simulink model "BoostPFCConverter"  (R2026a)
settings: Solver=ode23t  StopTime=0.05  MaxStep=1e-5  AbsTol=1e-3
PreLoadFcn:
  | BoostPFCDefaultInputParameters;
model workspace (MAT data in the model file):
  ConverterKey : string (value not decoded)
undefined symbols (not defined in the file): boostPFCController, boostPFCDesign, Rload_R, Vref
libraries: fl_lib x27, ee_lib x14, nesl_utility x14, ConverterLibrary x1
(part 2 of 2)

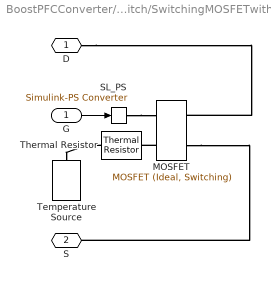
== system BoostPFCConverter/Boost PFC/BoostPFCVariant/DetailedModel/BoostSwitch/SwitchingMOSFETwithThermal ==
  G : Inport
  MOSFET : ee_lib/Semiconductors & Converters/MOSFET (Ideal, Switching)  PartSpecification="{\"CollectionId\":\"MW.SimscapeElectrical\",\"CollectionVersion\":\"1.0.0\",\"DatasetId\":\"Wolfspeed|C3M0015065K|\",\"DisplayName\":\"Wolfspeed:C3M0015065K\"}"  port_option=ee.enum.controlport.ps  Rds=0.015 % Datasheet derived Ohm  Goff=1.53846153846154e-09 % Datasheet derived S  Vth=2.3 % Wolfspeed XML derived V  diode_param=ee.enum.semiconductors.protectionDiode.external  diode_Vf=1.96 % Datasheet derived V  diode_Ron=0.007 % Wolfspeed XML derived Ohm  diode_Goff=1e-05 % Library default S  diode_C=50e-9 % Parameter not set F  diode_iRM=-235 % Parameter not set A  diode_iF=300 % Parameter not set A  diode_idot=-50 % Parameter not set A/us  diode_trr_param=ee.enum.converters.diodeReverseParam.trr_factor  diode_trr_factor=3 % Parameter not set  diode_trr=15 % Parameter not set us  diode_Qrr=1500 % Parameter not set s*uA  ids_specify=off  ids_priority=None  ids=0 A  ids_nominal_specify=off  ids_nominal_value=1  ids_nominal_unit=A  vds_specify=off  vds_priority=None  vds=0 V  vds_nominal_specify=off  vds_nominal_value=1  vds_nominal_unit=V  vgs_specify=off  vgs_priority=None  vgs=0 V  vgs_nominal_specify=off  vgs_nominal_value=1  vgs_nominal_unit=V  thermal_loss_option=ee.enum.converters.thermalLossOption.tabulated2d  Von_data=[-2.66 -2.44 -1.95 -1.414 -0.78 -0.41 -0.165 -0.082 -0.0343 0 0.037 0.078 0.179 0.43 0.83 1.68 2.597 3.5358 4.01;-2.83 -2.54 -1.975 -1.397 -0.75 -0.38 -0.155 -0.08 -0.03 0 0.034 0.067 0.16 0.39 0.76 1.549 2.4 3.26 3.72;-4.517 -4 -2.934 -1.965 -1 -0.51 -0.2048 -0.1018 -0.041 0 0.042 0.085 0.2 0.496 0.997 2.035 3.12 4.4 5.045;-5 -4.4 -3.2274 -2.1615 -1.1 -0.561 -0.22528 -0.11198 -0.0451 0 0.0462 0.0935 0.22 0.5456 1.0967 2.2385 3.432 4.84 5.5495] % Wolfspeed XML derived V  Tj=[-40 25 175 900] % Wolfspeed XML derived degC  Iout_data=[-225 -200 -150 -100 -50 -25 -10 -5 -2 0 2 5 10 25 50 100 150 200 225] % Wolfspeed XML derived A  tabulateWithVds=true  Eon_data=[0 9.96967576216216e-05 0.000145936917654886 0.000196497951068607 0.00019967532764657 0.000247335976316008 0.000304217502237006 0.000365133507991684;0 9.59855482079002e-05 0.000143792560765073 0.000194828655567568 0.000198273960318087 0.000249953531575884 0.000309139293804574 0.000373083909954262;0 9.79543049313929e-05 0.00014827399604158 0.000204722913230769 0.000208316887241164 0.000262226497397089 0.000326590011941788 0.000392096453887734;0 9.94356283409563e-05 0.000153658587442827 0.000209975271517672 0.000213824500004158 0.000271562927301455 0.000335992545829522 0.000402717496316008;0 0.000104407409862786 0.000161341516640333 0.000220474035093555 0.000224515725 0.000285141073596674 0.000352792173505198 0.000422853371376299] % Wolfspeed XML derived J  Eoff_data=[0 1.84408651719851e-05 4.70462491740572e-05 8.90430247881139e-05 9.1842809829051e-05 0.000147567719056776 0.000209864407870079 0.000278943613503315;0 2.00265752898881e-05 4.98845677374637e-05 9.33904774060557e-05 9.62908713839619e-05 0.000152525717421674 0.000215755778797141 0.000286903323875052;0 1.96758643514298e-05 5.11710664647741e-05 9.55627110851896e-05 9.8522154059884e-05 0.000155956102939287 0.000220242998240779 0.000292319989582884;0 1.96080415026937e-05 5.1490482059884e-05 9.66068334349875e-05 9.96145901933278e-05 0.000157442558060298 0.000223828680222752 0.000296440030520307;0 2.05884438265644e-05 5.40650061317862e-05 0.000101437175308835 0.000104595319920638 0.000165314685994405 0.000235020113767509 0.00031126203170431] % Wolfspeed XML derived J  Eon_data_3D=reshape([0;0;0;0;0;0;0;0;0;0;0;0;0;0;0;0;0;0;0;0;0;0;0;0;0;0;0;0;0;0;0;0;0;0;0;0;0;0;0;0;0;0;0;0;0;0;0;0;0;0;0;0;0;0;0;0;0;0;0;0;0;0;0;0;0;0;0;0;0;0;0;0;0;0;0;0;0;0;0;0;0;0;0;0;0;9.96967576216216e-05;9.59855482079002e-05;9.79543049313929e-05;9.94356283409563e-05;0.000104407409862786;0.000145936917654886;0.000143792560765073;0.00014827399604158;0.000153658587442827;0.000161341516640333;0.000196497951068607;0.000194828655567568;0.000204722913230769;0.000209975271517672;0.000220474035093555;0.00019967532764657;0.000198273960318087;0.000208316887241164;0.000213824500004158;0.000224515725;0.000247335976316008;0.000249953531575884;0.000262226497397089;0.000271562927301455;0.000285141073596674;0.000304217502237006;0.000309139293804574;0.000326590011941788;0.000335992545829522;0.000352792173505198;0.000365133507991684;0.000373083909954262;0.000392096453887734;0.000402717496316008;0.000422853371376299],[5 8 3]) % Wolfspeed XML derived J  Eoff_data_3D=reshape([0;0;0;0;0;0;0;0;0;0;0;0;0;0;0;0;0;0;0;0;0;0;0;0;0;0;0;0;0;0;0;0;0;0;0;0;0;0;0;0;0;0;0;0;0;0;0;0;0;0;0;0;0;0;0;0;0;0;0;0;0;0;0;0;0;0;0;0;0;0;0;0;0;0;0;0;0;0;0;0;0;0;0;0;0;1.84408651719851e-05;2.00265752898881e-05;1.96758643514298e-05;1.96080415026937e-05;2.05884438265644e-05;4.70462491740572e-05;4.98845677374637e-05;5.11710664647741e-05;5.1490482059884e-05;5.40650061317862e-05;8.90430247881139e-05;9.33904774060557e-05;9.55627110851896e-05;9.66068334349875e-05;0.000101437175308835;9.1842809829051e-05;9.62908713839619e-05;9.8522154059884e-05;9.96145901933278e-05;0.000104595319920638;0.000147567719056776;0.000152525717421674;0.000155956102939287;0.000157442558060298;0.000165314685994405;0.000209864407870079;0.000215755778797141;0.000220242998240779;0.000223828680222752;0.000235020113767509;0.000278943613503315;0.000286903323875052;0.000292319989582884;0.000296440030520307;0.00031126203170431],[5 8 3]) % Wolfspeed XML derived J  Tj_loss=[25 75 125 150 900] % Wolfspeed XML derived degC  Iout_data_loss=[0 12.8 26.4 38.4 39.2 51.2 62.4 74.4] % Wolfspeed XML derived A  Vds_loss=[-10 0 400] % Wolfspeed XML derived V  Eon_scalar=22.86e-3 % Parameter not set J  Eoff_scalar=17.14e-3 % Parameter not set J  Voff=300 % Parameter not set V  Iout_scalar=600 % Parameter not set A  useCurrentFromPreviousCycle=false % Parameter not set  useVoltageFromPreviousCycle=false % Parameter not set  diodeModelType=ee.enum.converters.diodeModelType.tabulated  diodeTableType=ee.enum.diode.tableType.VfMat  diode_ReverseIVType=ee.enum.diode.diodeReverseIV.constant  diode_IfMat=[.07, .12, .19, 1.75, 4.24, 7.32, 11.2; .16, .3, .72, 2.14, 4.02, 6.35, 9.12] % Parameter not set A  diode_VfMat=[0 2.87 3.94 4.34 5.07 5.76 6.58 7.12 7.53 7.697;0 2.68 3.54 3.9 4.55 5.26 6.12 6.72 7.18 7.38;0 2.31 3.11 3.45 4.06 4.72 5.61 6.24 6.76 6.987;0 2.079 2.799 3.105 3.654 4.248 5.049 5.616 6.084 6.3] % Wolfspeed XML derived V  diode_TjVec=[-40 25 175 900] % Wolfspeed XML derived degC  diode_VfVec=[.5, .7, .9, 1.3, 1.7, 2.1, 2.5] % Parameter not set V  diode_IfVec=[0 0.13 5 10 25 50 100 150 200 225] % Wolfspeed XML derived A  diode_IrMat=[1e-06, 2e-06, 5e-06, 1e-05, 2.5e-05, 5e-05, .0001; 2e-06, 5e-06, 1e-05, 4e-05, 8e-05, .0002, .0005] % Parameter not set A  diode_VrMat=[10, 100, 200, 250, 300, 325, 350; 10, 70, 160, 220, 270, 300, 320] % Parameter not set V  diode_VrVec=[10, 20, 40, 50, 70, 80, 100] % Parameter not set V  diode_IrVec=[1e-06, 2e-06, 5e-06, 1e-05, 2e-05, 5e-05, .0001] % Parameter not set A  diode_Vr=-600 % Parameter not set V  diode_Ls=150 % Parameter not set nH  diode_Erec=0.03 % Parameter not set J  diode_rec_loss_model=ee.enum.diode.reverseRecoveryModel.tabulated2d  diode_ErecVal=0 % Parameter not set J  diode_scaleWithIandV=true % Parameter not set  diode_ErecMat=[0 0;0 0] % Wolfspeed XML derived J  diodeErecMat3D=zeros(2, 3, 2) J  diode_TjrecVec=[25 35] % Wolfspeed XML derived degC  diode_IfrecVec=[0 10] % Wolfspeed XML derived A  diodeVrecVec=[0, 100] V  diode_IrecVal=10 % Parameter not set A  diode_VrecVal=10 % Wolfspeed XML derived V  diode_tFilter=1 / 1000 / 100 % Parameter not set s  separateThermalPortForDiode=false  thermal_network_parameterization=ee.enum.thermalNetworkTopology.external  Rth=[.03, .2] % Parameter not set K/W  Rth_Cauer=[0.040544078 0.111521813 0.073003418 0.124838849] % Wolfspeed XML derived K/W  Rth_Foster=[.08, .14, .22, .16] % Parameter not set K/W  thermal_mass_parameterization=ee.enum.thermalNetwork.thermalmass  thermal_mass=[3, 25] % Parameter not set J/K  thermal_mass_Cauer=[0.002121535 0.01054405 0.031037314 0.127325435] % Wolfspeed XML derived J/K  thermal_mass_Foster=[.001, .005, .05, .5] % Parameter not set J/K  thermal_time_constant=[.1, 5] % Parameter not set s  thermal_time_constant_Cauer=[.1, 1, 5] % Parameter not set s  thermal_time_constant_Foster=[7e-05, .0007, .01, .08] % Parameter not set s  thermal_mass_initial_temperatures=[25, 25] % Parameter not set degC  thermal_mass_initial_temperatures_Cauer=[25 25 25 25] % Wolfspeed XML derived degC  junction_thermal_mass=0.01 % Parameter not set J/K  Tvec_initial_Foster=[25, 25, 25, 25] % Parameter not set degC  RthDiode=[.03, .2] % Parameter not set K/W  RthCauerDiode=[0.04054 0.1115 0.073 0.1248] % Wolfspeed XML derived K/W  RthFosterDiode=[.03, .2] % Parameter not set K/W  thermalMassDiode=[3, 25] % Parameter not set J/K  thermalMassCauerDiode=[0.002122 0.01054 0.03104 0.1273] % Wolfspeed XML derived J/K  thermalMassFosterDiode=[33, 50] % Parameter not set J/K  thermalTauDiode=[.1, 5] % Parameter not set s  thermalTauCauerDiode=[.1, 1, 5] % Parameter not set s  thermalTauFosterDiode=[1, 10] % Parameter not set s  thermalMassInitTempDiode=[25, 25] % Parameter not set degC  thermalMassInitTempCauerDiode=[25 25 25 25] % Wolfspeed XML derived degC  junctionthermalMassDiode=0.1 % Parameter not set J/K  TVecInitialFosterDiode=[25, 25, 25, 25] % Parameter not set degC  no_thermal_network=0 % Parameter not set  mosfet_junction_temperature_specify=off  mosfet_junction_temperature_priority=None  mosfet_junction_temperature=simTemp_K K  mosfet_junction_temperature_nominal_specify=off  mosfet_junction_temperature_nominal_value=1  mosfet_junction_temperature_nominal_unit=degC  diode_junction_temperature_specify=off  diode_junction_temperature_priority=None  diode_junction_temperature=simTemp_K K  diode_junction_temperature_nominal_specify=off  diode_junction_temperature_nominal_value=1  diode_junction_temperature_nominal_unit=degC  Qj_specify=off  Qj_priority=None  Qj=0 W  Qj_nominal_specify=off  Qj_nominal_value=1  Qj_nominal_unit=W  accumulatedSwitchingLosses_specify=off  accumulatedSwitchingLosses_priority=None  accumulatedSwitchingLosses=0 J
      settings: AttributesFormatString=Wolfspeed:C3M0015065K
  SL_PS : nesl_utility/Simulink-PS Converter  PhysicalDomain=network_engine_domain  SubClassName=ps_input  LeftPortType=input  RightPortType=output  PseudoPeriodic=off  Frequencies=[]  NoiseDistribution=none  NoiseParameters=[]  Unit=1  AffineConversion=off  FilteringAndDerivatives=provide  SimscapeFilterOrder=1  InputFilterTimeConstant=0.001  UdotUserProvided=0
  Temperature Source : fl_lib/Thermal/Thermal Sources/Temperature Source  temperature=simTemp_K K
  Thermal Resistor : ee_lib/Passive/Thermal/Thermal Resistor  R=1e-3 K/W  T_specify=off  T_priority=None  T=0 K  T_nominal_specify=off  T_nominal_value=1  T_nominal_unit=K  Q_specify=off  Q_priority=None  Q=0 W  Q_nominal_specify=off  Q_nominal_value=1  Q_nominal_unit=W
  D : PMIOPort  Side=Left
  S : PMIOPort  Port=2  Side=Right
  wires:
  G/1 -> SL_PS/1
  connections:
  Thermal Resistor/LConn1 -- Temperature Source/LConn1
  MOSFET/LConn2 -- Thermal Resistor/RConn1
  MOSFET/RConn2 -- S/RConn1
  D/RConn1 -- MOSFET/RConn1
  SL_PS/RConn1 -- MOSFET/LConn1

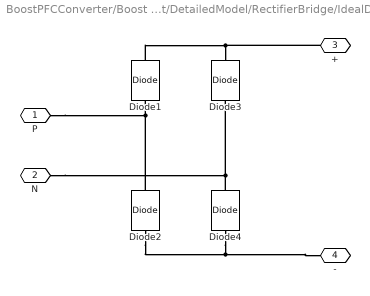
== system BoostPFCConverter/Boost PFC/BoostPFCVariant/DetailedModel/RectifierBridge/IdealDiode ==
  Diode{1..4} (4 alike) : fl_lib/Electrical/Electrical Elements/Diode  Vf=VfRect_SI V  Ron=RdRect_SI Ohm  Goff=GdRect_SI 1/Ohm  i_specify=off  i_priority=None  i=0 A  i_nominal_specify=off  i_nominal_value=1  i_nominal_unit=A  v_specify=off  v_priority=None  v=0 V  v_nominal_specify=off  v_nominal_value=1  v_nominal_unit=V
  P : PMIOPort  Side=Left
  N : PMIOPort  Port=2  Side=Left
  + : PMIOPort  Port=3  Side=Right
  - : PMIOPort  Port=4  Side=Right
  connections:
  Diode2/LConn1 -- -/RConn1 -- Diode4/LConn1
  Diode4/RConn1 -- N/RConn1 -- Diode3/LConn1
  Diode2/RConn1 -- P/RConn1 -- Diode1/LConn1
  Diode1/RConn1 -- +/RConn1 -- Diode3/RConn1

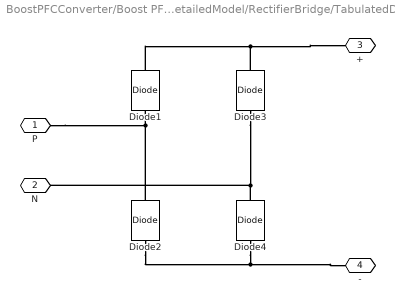
== system BoostPFCConverter/Boost PFC/BoostPFCVariant/DetailedModel/RectifierBridge/TabulatedDiode ==
  Diode1 : ee_lib/Semiconductors & Converters/Diode  PartSpecification="{\"CollectionId\":\"MW.SimscapeElectrical\",\"CollectionVersion\":\"1.0.0\",\"DatasetId\":\"Infineon|IDW80C65D1|simscape.electrical.diode\",\"DisplayName\":\"Infineon:IDW80C65D1\"}"  ModelType=ee.enum.diode.modelType.tabulated  TableType=ee.enum.diode.tableType.IfMat  IfMat=[0.0001 0.0001 0.1601 0.6065 1.9426 5.4603 12.2546 21.9425 34.4556 49.1982 64.7538 83.3404;0.3114 0.8503 2.3479 5.2232 9.8335 15.9488 23.5801 32.5233 43.1998 54.3228 66.653 79.8979] % Datasheet derived A  VfMat=[.9, 1.15, 1.25, 1.5, 1.75, 2.17, 2.6, 2.85; .58, .68, .75, 1.1, 1.38, 1.77, 2.27, 2.7] % Parameter not set V  TjVec=[25 175] % Datasheet derived degC  VfVec=[0.3258 0.4465 0.5672 0.6878 0.8085 0.9292 1.0498 1.1705 1.2912 1.4118 1.5325 1.6532] % Datasheet derived V  IfVec=[.1, .2, .5, 1, 2, 4, 7, 10] % Parameter not set A  IrMat=[1e-06, 2e-06, 5e-06, 1e-05, 2.5e-05, 5e-05, .0001; 2e-06, 5e-06, 1e-05, 4e-05, 8e-05, .0002, .0005] % Parameter not set A  VrMat=[10, 100, 200, 250, 300, 325, 350; 10, 70, 160, 220, 270, 300, 320] % Parameter not set V  VrVec=[10, 20, 40, 50, 70, 80, 100] % Parameter not set V  IrVec=[1e-06, 2e-06, 5e-06, 1e-05, 2e-05, 5e-05, .0001] % Parameter not set A  Vf=0.6 % Parameter not set V  Ron=0.3 % Parameter not set Ohm  Goff=1e-08 % Parameter not set S  prmExp=ee.enum.diode.expParam.useTwo  I12=[.0137, .545] % Parameter not set A  V12=[.6, .7] % Parameter not set V  RS=0 % Parameter not set Ohm  Tmeas=298.15 % Parameter not set K  IS=1e-12 % Parameter not set A  ec=1 % Parameter not set  I1=0.0137 % Parameter not set A  V1=0.6 % Parameter not set V  N_series=1 % Parameter not set  N_parallel=1 % Parameter not set  ZenerEnable=false % Parameter not set  Rz=0.3 % Parameter not set Ohm  BV=inf % Parameter not set V  C_param=ee.enum.diode.capParam.fixed  CJ=0 % Parameter not set pF  CJ0=5 % Parameter not set pF  Vvec=[.1, 10, 100] % Parameter not set V  Cvec=[3.5, 1, .4] % Parameter not set pF  VJ=1 % Parameter not set V  Mgrad=0.5 % Parameter not set  FC=0.5 % Parameter not set  Q_param=ee.enum.diode.recoveryParam.off  iRM=-7.15 % Parameter not set A  iF=4 % Parameter not set A  didt=-750 % Parameter not set A/us  trr_factor=3 % Parameter not set  trr=115 % Parameter not set ns  Qrr=150 % Parameter not set nA*s  Vr=-600 % Parameter not set V  Ls=150 % Parameter not set nH  Erec=0.03 % Parameter not set J  TT=50 % Parameter not set ns  tau=100 % Parameter not set ns  T_param=ee.enum.diode.temperatureParam.off  Tdevice=simTemp_K K  I1_T2=0.245 % Parameter not set A  V1_T2=0.5 % Parameter not set V  IS_T2=1.25e-7 % Parameter not set A  Tmeas2=125 % Parameter not set degC  XTI_param=ee.enum.diode.xtiParam.pn  XTI=3 % Parameter not set  EG_param=ee.enum.diode.egapParam.material_si  EG=1.11 % Parameter not set eV  dBVdT=0 % Parameter not set V/K  enable_fault_input=simscape.enum.onoff.off  i_specify=off  i_priority=None  i=0 A  i_nominal_specify=off  i_nominal_value=1  i_nominal_unit=A  v_specify=off  v_priority=None  v=0 V  v_nominal_specify=off  v_nominal_value=1  v_nominal_unit=V  v_capacitor_specify=off  v_capacitor_priority=None  v_capacitor=0 V  v_capacitor_nominal_specify=off  v_capacitor_nominal_value=1  v_capacitor_nominal_unit=V  Qj_specify=off  Qj_priority=High  Qj=0 C  Qj_nominal_specify=off  Qj_nominal_value=1  Qj_nominal_unit=C  i_diode_specify=off  i_diode_priority=None  i_diode=0 A  i_diode_nominal_specify=off  i_diode_nominal_value=1  i_diode_nominal_unit=A  v_diode_specify=off  v_diode_priority=None  v_diode=0 V  v_diode_nominal_specify=off  v_diode_nominal_value=1  v_diode_nominal_unit=V  i_capacitor_specify=off  i_capacitor_priority=None  i_capacitor=0 A  i_capacitor_nominal_specify=off  i_capacitor_nominal_value=1  i_capacitor_nominal_unit=A  fidelity_level=ee.enum.diode.fidelity.includeChargeDyn  rec_loss_model=ee.enum.diode.reverseRecoveryModel.fixed  ErecVal=0 % Parameter not set J  scaleWithIandV=true % Parameter not set  ErecMat=zeros(2, 3) % Parameter not set J  ErecMat3D=zeros(2, 3, 2) J  TjrecVec=[298.15, 398.15] % Parameter not set K  IfrecVec=[.1, 1, 10] % Parameter not set A  IrecVal=10 % Parameter not set A  VrecVal=10 % Parameter not set V  VrecVec=[0, 100] V  tFilter=1 / 1000 / 100 % Parameter not set s  thermal_network_parameterization=ee.enum.thermalNetworkTopology.junctionCase  Rth=[0, 10] % Parameter not set K/W  Rth_Cauer=[1, 3, 10] % Parameter not set K/W  Rth_Foster=[.08, .14, .22, .16] % Parameter not set K/W  thermal_mass_parameterization=ee.enum.thermalNetwork.timeconstant  thermal_mass=[0, 1] % Parameter not set J/K  thermal_mass_Cauer=[.1, .3, 1] % Parameter not set J/K  thermal_mass_Foster=[.001, .005, .05, .5] % Parameter not set J/K  thermal_time_constant=[0, 10] % Parameter not set s  thermal_time_constant_Cauer=[1, 3, 10] % Parameter not set s  thermal_time_constant_Foster=[7e-05, .0007, .01, .08] % Parameter not set s  thermal_mass_initial_temperatures=[25, 25] % Parameter not set degC  thermal_mass_initial_temperatures_Cauer=[25, 25, 25] % Parameter not set degC  junction_thermal_mass=0.01 % Parameter not set J/K  Tvec_initial_Foster=[25, 25, 25, 25] % Parameter not set degC  no_thermal_network=0 % Parameter not set  junction_temperature_specify=off  junction_temperature_priority=None  junction_temperature=25 degC  junction_temperature_nominal_specify=off  junction_temperature_nominal_value=1  junction_temperature_nominal_unit=degC
      settings: AttributesFormatString=Infineon:IDW80C65D1
  Diode2 : ee_lib/Semiconductors & Converters/Diode  ModelType=ee.enum.diode.modelType.tabulated  TableType=ee.enum.diode.tableType.IfMat  IfMat=[0.0001 0.0001 0.1601 0.6065 1.9426 5.4603 12.2546 21.9425 34.4556 49.1982 64.7538 83.3404;0.3114 0.8503 2.3479 5.2232 9.8335 15.9488 23.5801 32.5233 43.1998 54.3228 66.653 79.8979] % Datasheet derived A  VfMat=[.9, 1.15, 1.25, 1.5, 1.75, 2.17, 2.6, 2.85; .58, .68, .75, 1.1, 1.38, 1.77, 2.27, 2.7] % Parameter not set V  TjVec=[25 175] % Datasheet derived degC  VfVec=[0.3258 0.4465 0.5672 0.6878 0.8085 0.9292 1.0498 1.1705 1.2912 1.4118 1.5325 1.6532] % Datasheet derived V  IfVec=[.1, .2, .5, 1, 2, 4, 7, 10] % Parameter not set A  IrMat=[1e-06, 2e-06, 5e-06, 1e-05, 2.5e-05, 5e-05, .0001; 2e-06, 5e-06, 1e-05, 4e-05, 8e-05, .0002, .0005] % Parameter not set A  VrMat=[10, 100, 200, 250, 300, 325, 350; 10, 70, 160, 220, 270, 300, 320] % Parameter not set V  VrVec=[10, 20, 40, 50, 70, 80, 100] % Parameter not set V  IrVec=[1e-06, 2e-06, 5e-06, 1e-05, 2e-05, 5e-05, .0001] % Parameter not set A  Vf=0.6 % Parameter not set V  Ron=0.3 % Parameter not set Ohm  Goff=1e-08 % Parameter not set S  prmExp=ee.enum.diode.expParam.useTwo  I12=[.0137, .545] % Parameter not set A  V12=[.6, .7] % Parameter not set V  RS=0 % Parameter not set Ohm  Tmeas=298.15 % Parameter not set K  IS=1e-12 % Parameter not set A  ec=1 % Parameter not set  I1=0.0137 % Parameter not set A  V1=0.6 % Parameter not set V  N_series=1 % Parameter not set  N_parallel=1 % Parameter not set  ZenerEnable=false % Parameter not set  Rz=0.3 % Parameter not set Ohm  BV=inf % Parameter not set V  C_param=ee.enum.diode.capParam.fixed  CJ=0 % Parameter not set pF  CJ0=5 % Parameter not set pF  Vvec=[.1, 10, 100] % Parameter not set V  Cvec=[3.5, 1, .4] % Parameter not set pF  VJ=1 % Parameter not set V  Mgrad=0.5 % Parameter not set  FC=0.5 % Parameter not set  Q_param=ee.enum.diode.recoveryParam.off  iRM=-7.15 % Parameter not set A  iF=4 % Parameter not set A  didt=-750 % Parameter not set A/us  trr_factor=3 % Parameter not set  trr=115 % Parameter not set ns  Qrr=150 % Parameter not set nA*s  Vr=-600 % Parameter not set V  Ls=150 % Parameter not set nH  Erec=0.03 % Parameter not set J  TT=50 % Parameter not set ns  tau=100 % Parameter not set ns  T_param=ee.enum.diode.temperatureParam.off  Tdevice=simTemp_K K  I1_T2=0.245 % Parameter not set A  V1_T2=0.5 % Parameter not set V  IS_T2=1.25e-7 % Parameter not set A  Tmeas2=125 % Parameter not set degC  XTI_param=ee.enum.diode.xtiParam.pn  XTI=3 % Parameter not set  EG_param=ee.enum.diode.egapParam.material_si  EG=1.11 % Parameter not set eV  dBVdT=0 % Parameter not set V/K  enable_fault_input=simscape.enum.onoff.off  i_specify=off  i_priority=None  i=0 A  i_nominal_specify=off  i_nominal_value=1  i_nominal_unit=A  v_specify=off  v_priority=None  v=0 V  v_nominal_specify=off  v_nominal_value=1  v_nominal_unit=V  v_capacitor_specify=off  v_capacitor_priority=None  v_capacitor=0 V  v_capacitor_nominal_specify=off  v_capacitor_nominal_value=1  v_capacitor_nominal_unit=V  Qj_specify=off  Qj_priority=High  Qj=0 C  Qj_nominal_specify=off  Qj_nominal_value=1  Qj_nominal_unit=C  i_diode_specify=off  i_diode_priority=None  i_diode=0 A  i_diode_nominal_specify=off  i_diode_nominal_value=1  i_diode_nominal_unit=A  v_diode_specify=off  v_diode_priority=None  v_diode=0 V  v_diode_nominal_specify=off  v_diode_nominal_value=1  v_diode_nominal_unit=V  i_capacitor_specify=off  i_capacitor_priority=None  i_capacitor=0 A  i_capacitor_nominal_specify=off  i_capacitor_nominal_value=1  i_capacitor_nominal_unit=A  fidelity_level=ee.enum.diode.fidelity.includeChargeDyn  rec_loss_model=ee.enum.diode.reverseRecoveryModel.fixed  ErecVal=0 % Parameter not set J  scaleWithIandV=true % Parameter not set  ErecMat=zeros(2, 3) % Parameter not set J  ErecMat3D=zeros(2, 3, 2) J  TjrecVec=[298.15, 398.15] % Parameter not set K  IfrecVec=[.1, 1, 10] % Parameter not set A  IrecVal=10 % Parameter not set A  VrecVal=10 % Parameter not set V  VrecVec=[0, 100] V  tFilter=1 / 1000 / 100 % Parameter not set s  thermal_network_parameterization=ee.enum.thermalNetworkTopology.junctionCase  Rth=[0, 10] % Parameter not set K/W  Rth_Cauer=[1, 3, 10] % Parameter not set K/W  Rth_Foster=[.08, .14, .22, .16] % Parameter not set K/W  thermal_mass_parameterization=ee.enum.thermalNetwork.timeconstant  thermal_mass=[0, 1] % Parameter not set J/K  thermal_mass_Cauer=[.1, .3, 1] % Parameter not set J/K  thermal_mass_Foster=[.001, .005, .05, .5] % Parameter not set J/K  thermal_time_constant=[0, 10] % Parameter not set s  thermal_time_constant_Cauer=[1, 3, 10] % Parameter not set s  thermal_time_constant_Foster=[7e-05, .0007, .01, .08] % Parameter not set s  thermal_mass_initial_temperatures=[25, 25] % Parameter not set degC  thermal_mass_initial_temperatures_Cauer=[25, 25, 25] % Parameter not set degC  junction_thermal_mass=0.01 % Parameter not set J/K  Tvec_initial_Foster=[25, 25, 25, 25] % Parameter not set degC  no_thermal_network=0 % Parameter not set  junction_temperature_specify=off  junction_temperature_priority=None  junction_temperature=25 degC  junction_temperature_nominal_specify=off  junction_temperature_nominal_value=1  junction_temperature_nominal_unit=degC
  Diode3 : ee_lib/Semiconductors & Converters/Diode  ModelType=ee.enum.diode.modelType.tabulated  TableType=ee.enum.diode.tableType.IfMat  IfMat=[0.0001 0.0001 0.1601 0.6065 1.9426 5.4603 12.2546 21.9425 34.4556 49.1982 64.7538 83.3404;0.3114 0.8503 2.3479 5.2232 9.8335 15.9488 23.5801 32.5233 43.1998 54.3228 66.653 79.8979] % Datasheet derived A  VfMat=[.9, 1.15, 1.25, 1.5, 1.75, 2.17, 2.6, 2.85; .58, .68, .75, 1.1, 1.38, 1.77, 2.27, 2.7] % Parameter not set V  TjVec=[25 175] % Datasheet derived degC  VfVec=[0.3258 0.4465 0.5672 0.6878 0.8085 0.9292 1.0498 1.1705 1.2912 1.4118 1.5325 1.6532] % Datasheet derived V  IfVec=[.1, .2, .5, 1, 2, 4, 7, 10] % Parameter not set A  IrMat=[1e-06, 2e-06, 5e-06, 1e-05, 2.5e-05, 5e-05, .0001; 2e-06, 5e-06, 1e-05, 4e-05, 8e-05, .0002, .0005] % Parameter not set A  VrMat=[10, 100, 200, 250, 300, 325, 350; 10, 70, 160, 220, 270, 300, 320] % Parameter not set V  VrVec=[10, 20, 40, 50, 70, 80, 100] % Parameter not set V  IrVec=[1e-06, 2e-06, 5e-06, 1e-05, 2e-05, 5e-05, .0001] % Parameter not set A  Vf=0.6 % Parameter not set V  Ron=0.3 % Parameter not set Ohm  Goff=1e-08 % Parameter not set S  prmExp=ee.enum.diode.expParam.useTwo  I12=[.0137, .545] % Parameter not set A  V12=[.6, .7] % Parameter not set V  RS=0 % Parameter not set Ohm  Tmeas=298.15 % Parameter not set K  IS=1e-12 % Parameter not set A  ec=1 % Parameter not set  I1=0.0137 % Parameter not set A  V1=0.6 % Parameter not set V  N_series=1 % Parameter not set  N_parallel=1 % Parameter not set  ZenerEnable=false % Parameter not set  Rz=0.3 % Parameter not set Ohm  BV=inf % Parameter not set V  C_param=ee.enum.diode.capParam.fixed  CJ=0 % Parameter not set pF  CJ0=5 % Parameter not set pF  Vvec=[.1, 10, 100] % Parameter not set V  Cvec=[3.5, 1, .4] % Parameter not set pF  VJ=1 % Parameter not set V  Mgrad=0.5 % Parameter not set  FC=0.5 % Parameter not set  Q_param=ee.enum.diode.recoveryParam.off  iRM=-7.15 % Parameter not set A  iF=4 % Parameter not set A  didt=-750 % Parameter not set A/us  trr_factor=3 % Parameter not set  trr=115 % Parameter not set ns  Qrr=150 % Parameter not set nA*s  Vr=-600 % Parameter not set V  Ls=150 % Parameter not set nH  Erec=0.03 % Parameter not set J  TT=50 % Parameter not set ns  tau=100 % Parameter not set ns  T_param=ee.enum.diode.temperatureParam.off  Tdevice=simTemp_K K  I1_T2=0.245 % Parameter not set A  V1_T2=0.5 % Parameter not set V  IS_T2=1.25e-7 % Parameter not set A  Tmeas2=125 % Parameter not set degC  XTI_param=ee.enum.diode.xtiParam.pn  XTI=3 % Parameter not set  EG_param=ee.enum.diode.egapParam.material_si  EG=1.11 % Parameter not set eV  dBVdT=0 % Parameter not set V/K  enable_fault_input=simscape.enum.onoff.off  i_specify=off  i_priority=None  i=0 A  i_nominal_specify=off  i_nominal_value=1  i_nominal_unit=A  v_specify=off  v_priority=None  v=0 V  v_nominal_specify=off  v_nominal_value=1  v_nominal_unit=V  v_capacitor_specify=off  v_capacitor_priority=None  v_capacitor=0 V  v_capacitor_nominal_specify=off  v_capacitor_nominal_value=1  v_capacitor_nominal_unit=V  Qj_specify=off  Qj_priority=High  Qj=0 C  Qj_nominal_specify=off  Qj_nominal_value=1  Qj_nominal_unit=C  i_diode_specify=off  i_diode_priority=None  i_diode=0 A  i_diode_nominal_specify=off  i_diode_nominal_value=1  i_diode_nominal_unit=A  v_diode_specify=off  v_diode_priority=None  v_diode=0 V  v_diode_nominal_specify=off  v_diode_nominal_value=1  v_diode_nominal_unit=V  i_capacitor_specify=off  i_capacitor_priority=None  i_capacitor=0 A  i_capacitor_nominal_specify=off  i_capacitor_nominal_value=1  i_capacitor_nominal_unit=A  fidelity_level=ee.enum.diode.fidelity.includeChargeDyn  rec_loss_model=ee.enum.diode.reverseRecoveryModel.fixed  ErecVal=0 % Parameter not set J  scaleWithIandV=true % Parameter not set  ErecMat=zeros(2, 3) % Parameter not set J  ErecMat3D=zeros(2, 3, 2) J  TjrecVec=[298.15, 398.15] % Parameter not set K  IfrecVec=[.1, 1, 10] % Parameter not set A  IrecVal=10 % Parameter not set A  VrecVal=10 % Parameter not set V  VrecVec=[0, 100] V  tFilter=1 / 1000 / 100 % Parameter not set s  thermal_network_parameterization=ee.enum.thermalNetworkTopology.junctionCase  Rth=[0, 10] % Parameter not set K/W  Rth_Cauer=[1, 3, 10] % Parameter not set K/W  Rth_Foster=[.08, .14, .22, .16] % Parameter not set K/W  thermal_mass_parameterization=ee.enum.thermalNetwork.timeconstant  thermal_mass=[0, 1] % Parameter not set J/K  thermal_mass_Cauer=[.1, .3, 1] % Parameter not set J/K  thermal_mass_Foster=[.001, .005, .05, .5] % Parameter not set J/K  thermal_time_constant=[0, 10] % Parameter not set s  thermal_time_constant_Cauer=[1, 3, 10] % Parameter not set s  thermal_time_constant_Foster=[7e-05, .0007, .01, .08] % Parameter not set s  thermal_mass_initial_temperatures=[25, 25] % Parameter not set degC  thermal_mass_initial_temperatures_Cauer=[25, 25, 25] % Parameter not set degC  junction_thermal_mass=0.01 % Parameter not set J/K  Tvec_initial_Foster=[25, 25, 25, 25] % Parameter not set degC  no_thermal_network=0 % Parameter not set  junction_temperature_specify=off  junction_temperature_priority=None  junction_temperature=25 degC  junction_temperature_nominal_specify=off  junction_temperature_nominal_value=1  junction_temperature_nominal_unit=degC
  Diode4 : ee_lib/Semiconductors & Converters/Diode  ModelType=ee.enum.diode.modelType.tabulated  TableType=ee.enum.diode.tableType.IfMat  IfMat=[0.0001 0.0001 0.1601 0.6065 1.9426 5.4603 12.2546 21.9425 34.4556 49.1982 64.7538 83.3404;0.3114 0.8503 2.3479 5.2232 9.8335 15.9488 23.5801 32.5233 43.1998 54.3228 66.653 79.8979] % Datasheet derived A  VfMat=[.9, 1.15, 1.25, 1.5, 1.75, 2.17, 2.6, 2.85; .58, .68, .75, 1.1, 1.38, 1.77, 2.27, 2.7] % Parameter not set V  TjVec=[25 175] % Datasheet derived degC  VfVec=[0.3258 0.4465 0.5672 0.6878 0.8085 0.9292 1.0498 1.1705 1.2912 1.4118 1.5325 1.6532] % Datasheet derived V  IfVec=[.1, .2, .5, 1, 2, 4, 7, 10] % Parameter not set A  IrMat=[1e-06, 2e-06, 5e-06, 1e-05, 2.5e-05, 5e-05, .0001; 2e-06, 5e-06, 1e-05, 4e-05, 8e-05, .0002, .0005] % Parameter not set A  VrMat=[10, 100, 200, 250, 300, 325, 350; 10, 70, 160, 220, 270, 300, 320] % Parameter not set V  VrVec=[10, 20, 40, 50, 70, 80, 100] % Parameter not set V  IrVec=[1e-06, 2e-06, 5e-06, 1e-05, 2e-05, 5e-05, .0001] % Parameter not set A  Vf=0.6 % Parameter not set V  Ron=0.3 % Parameter not set Ohm  Goff=1e-08 % Parameter not set S  prmExp=ee.enum.diode.expParam.useTwo  I12=[.0137, .545] % Parameter not set A  V12=[.6, .7] % Parameter not set V  RS=0 % Parameter not set Ohm  Tmeas=298.15 % Parameter not set K  IS=1e-12 % Parameter not set A  ec=1 % Parameter not set  I1=0.0137 % Parameter not set A  V1=0.6 % Parameter not set V  N_series=1 % Parameter not set  N_parallel=1 % Parameter not set  ZenerEnable=false % Parameter not set  Rz=0.3 % Parameter not set Ohm  BV=inf % Parameter not set V  C_param=ee.enum.diode.capParam.fixed  CJ=0 % Parameter not set pF  CJ0=5 % Parameter not set pF  Vvec=[.1, 10, 100] % Parameter not set V  Cvec=[3.5, 1, .4] % Parameter not set pF  VJ=1 % Parameter not set V  Mgrad=0.5 % Parameter not set  FC=0.5 % Parameter not set  Q_param=ee.enum.diode.recoveryParam.off  iRM=-7.15 % Parameter not set A  iF=4 % Parameter not set A  didt=-750 % Parameter not set A/us  trr_factor=3 % Parameter not set  trr=115 % Parameter not set ns  Qrr=150 % Parameter not set nA*s  Vr=-600 % Parameter not set V  Ls=150 % Parameter not set nH  Erec=0.03 % Parameter not set J  TT=50 % Parameter not set ns  tau=100 % Parameter not set ns  T_param=ee.enum.diode.temperatureParam.off  Tdevice=simTemp_K K  I1_T2=0.245 % Parameter not set A  V1_T2=0.5 % Parameter not set V  IS_T2=1.25e-7 % Parameter not set A  Tmeas2=125 % Parameter not set degC  XTI_param=ee.enum.diode.xtiParam.pn  XTI=3 % Parameter not set  EG_param=ee.enum.diode.egapParam.material_si  EG=1.11 % Parameter not set eV  dBVdT=0 % Parameter not set V/K  enable_fault_input=simscape.enum.onoff.off  i_specify=off  i_priority=None  i=0 A  i_nominal_specify=off  i_nominal_value=1  i_nominal_unit=A  v_specify=off  v_priority=None  v=0 V  v_nominal_specify=off  v_nominal_value=1  v_nominal_unit=V  v_capacitor_specify=off  v_capacitor_priority=None  v_capacitor=0 V  v_capacitor_nominal_specify=off  v_capacitor_nominal_value=1  v_capacitor_nominal_unit=V  Qj_specify=off  Qj_priority=High  Qj=0 C  Qj_nominal_specify=off  Qj_nominal_value=1  Qj_nominal_unit=C  i_diode_specify=off  i_diode_priority=None  i_diode=0 A  i_diode_nominal_specify=off  i_diode_nominal_value=1  i_diode_nominal_unit=A  v_diode_specify=off  v_diode_priority=None  v_diode=0 V  v_diode_nominal_specify=off  v_diode_nominal_value=1  v_diode_nominal_unit=V  i_capacitor_specify=off  i_capacitor_priority=None  i_capacitor=0 A  i_capacitor_nominal_specify=off  i_capacitor_nominal_value=1  i_capacitor_nominal_unit=A  fidelity_level=ee.enum.diode.fidelity.includeChargeDyn  rec_loss_model=ee.enum.diode.reverseRecoveryModel.fixed  ErecVal=0 % Parameter not set J  scaleWithIandV=true % Parameter not set  ErecMat=zeros(2, 3) % Parameter not set J  ErecMat3D=zeros(2, 3, 2) J  TjrecVec=[298.15, 398.15] % Parameter not set K  IfrecVec=[.1, 1, 10] % Parameter not set A  IrecVal=10 % Parameter not set A  VrecVal=10 % Parameter not set V  VrecVec=[0, 100] V  tFilter=1 / 1000 / 100 % Parameter not set s  thermal_network_parameterization=ee.enum.thermalNetworkTopology.junctionCase  Rth=[0, 10] % Parameter not set K/W  Rth_Cauer=[1, 3, 10] % Parameter not set K/W  Rth_Foster=[.08, .14, .22, .16] % Parameter not set K/W  thermal_mass_parameterization=ee.enum.thermalNetwork.timeconstant  thermal_mass=[0, 1] % Parameter not set J/K  thermal_mass_Cauer=[.1, .3, 1] % Parameter not set J/K  thermal_mass_Foster=[.001, .005, .05, .5] % Parameter not set J/K  thermal_time_constant=[0, 10] % Parameter not set s  thermal_time_constant_Cauer=[1, 3, 10] % Parameter not set s  thermal_time_constant_Foster=[7e-05, .0007, .01, .08] % Parameter not set s  thermal_mass_initial_temperatures=[25, 25] % Parameter not set degC  thermal_mass_initial_temperatures_Cauer=[25, 25, 25] % Parameter not set degC  junction_thermal_mass=0.01 % Parameter not set J/K  Tvec_initial_Foster=[25, 25, 25, 25] % Parameter not set degC  no_thermal_network=0 % Parameter not set  junction_temperature_specify=off  junction_temperature_priority=None  junction_temperature=25 degC  junction_temperature_nominal_specify=off  junction_temperature_nominal_value=1  junction_temperature_nominal_unit=degC
  P : PMIOPort  Side=Left
  N : PMIOPort  Port=2  Side=Left
  + : PMIOPort  Port=3  Side=Right
  - : PMIOPort  Port=4  Side=Right
  connections:
  Diode1/RConn1 -- +/RConn1 -- Diode3/RConn1
  Diode2/LConn1 -- -/RConn1 -- Diode4/LConn1
  Diode3/LConn1 -- Diode4/RConn1 -- N/RConn1
  Diode2/RConn1 -- P/RConn1 -- Diode1/LConn1
